simulink model "Ten_phase_nine_leg_relocated_L3_L7"  (R2025b)
settings: Solver=VariableStepAuto  StartTime=0.0  StopTime=0.05  FixedStep=1e-6  MaxStep=1e-6  RelTol=1e-4
values from neighbouring files (symbols this model uses):
  bias_current = 5    [parameters_for_AMB_topology.m]
  half_SW_Ts = SW_Ts*0.5    (= 2.5e-05)    [parameters_for_AMB_topology.m]
  K_i = 2*pi*f_c*R_value/U_dc    (= 47.1238898038)    [parameters_for_AMB_topology.m]
  K_p = 2*pi*f_c*L_value/U_dc    (= 0.0235619449019)    [parameters_for_AMB_topology.m]
  R_value = 1    [parameters_for_AMB_topology.m]
  SW_Ts = 1/(SW_frequency)    (= 5e-05)    [parameters_for_AMB_topology.m]
libraries: fl_lib x61, simulink x39, nesl_utility x29, eeGeneralControl x28, ee_lib x19
(part 1 of 4)
settings Model: SimulationMode=accelerator  Creator=ubuntu  LastModifiedBy=ubuntu

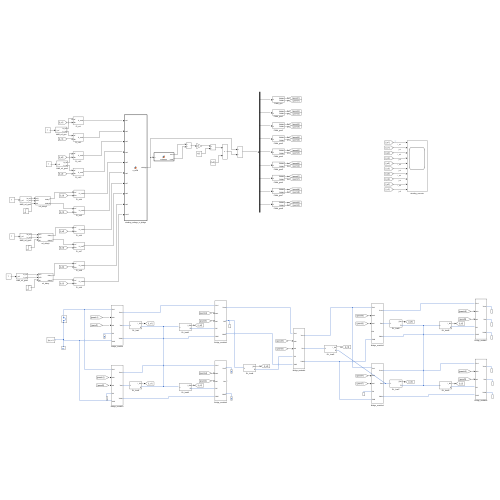
[thumbnail: Simulink's stored preview of the top-level diagram]
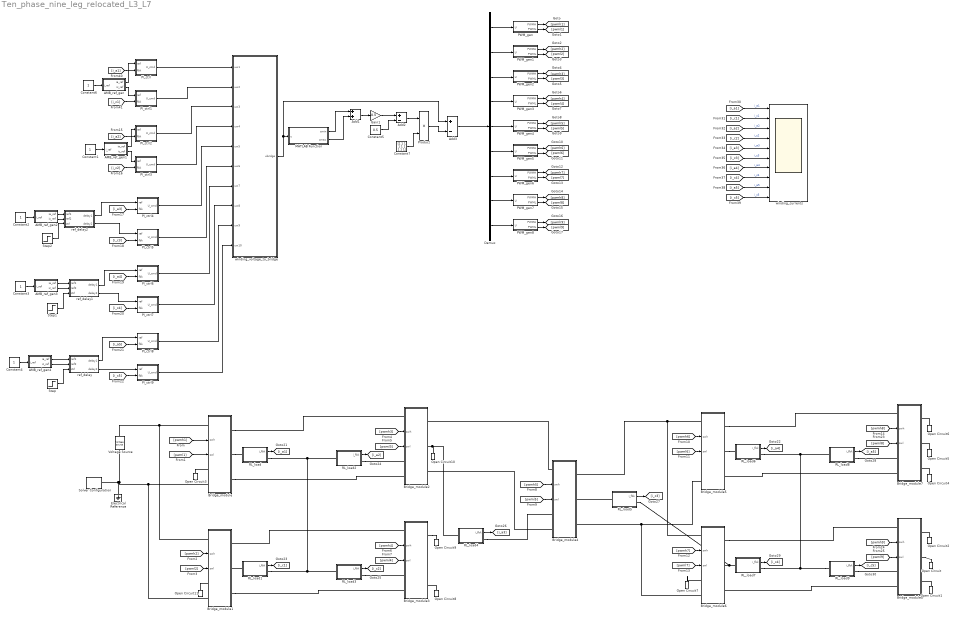
== system Ten_phase_nine_leg_relocated_L3_L7 ==
  AMB_ref_gen : Subsystem
  AMB_ref_gen1 : Subsystem
  AMB_ref_gen2 : Subsystem
  AMB_ref_gen3 : Subsystem
  AMB_ref_gen4 : Subsystem
  Add1 : Sum
  Add2 : Sum  Inputs=+-
  Add3 : Sum  Inputs=+-
  Bridge_module : Subsystem
      settings: PortSchema="{\"entries\":[{\"content\":{\"sides\":[{\"content\":{\"connectorIds\":[\"LConn1\",\"In1\",\"In2\",\"LConn2\",\"LConn3\"]},\"type\":\"ConnectorPlacement.EquallySpacedRectSide\",\"uuid\":\"d53b2940-a672-44eb-b8dc-5a9e6180756a\"},{\"content\":{\"connectorIds\":[\"RConn1\",\"RConn2\",\"RConn3\"],\"side\":\"RIGHT\"},\"type\":\"ConnectorPlacement.EquallySpacedRectSide\",\"uuid\":\"c4e7a2ca-919a-44db-8da7-3bac39d44d51\"},{\"content\":{\"side\":\"TOP\"},\"type\":\"ConnectorPlacement.EquallySpacedRectSide\",\"uuid\":\"b6113aa5-412c-49ab-b296-5158e67c3ca8\"}]},\"type\":\"ConnectorPlacement.EquallySpacedConnector\",\"uuid\":\"7447e388-299b-4a6a-b1b3-3d6a05a16289\"}],\"packageUris\":[\"http://schema.mathworks.com/mf0/Connector/R2020b\"],\"version\":\"1.0\"}"
  Bridge_module1 : Subsystem
      settings: PortSchema="{\"entries\":[{\"content\":{\"sides\":[{\"content\":{\"connectorIds\":[\"LConn1\",\"In1\",\"In2\",\"LConn2\",\"LConn3\"]},\"type\":\"ConnectorPlacement.EquallySpacedRectSide\",\"uuid\":\"d53b2940-a672-44eb-b8dc-5a9e6180756a\"},{\"content\":{\"connectorIds\":[\"RConn1\",\"RConn2\",\"RConn3\"],\"side\":\"RIGHT\"},\"type\":\"ConnectorPlacement.EquallySpacedRectSide\",\"uuid\":\"c4e7a2ca-919a-44db-8da7-3bac39d44d51\"},{\"content\":{\"side\":\"TOP\"},\"type\":\"ConnectorPlacement.EquallySpacedRectSide\",\"uuid\":\"b6113aa5-412c-49ab-b296-5158e67c3ca8\"}]},\"type\":\"ConnectorPlacement.EquallySpacedConnector\",\"uuid\":\"7447e388-299b-4a6a-b1b3-3d6a05a16289\"}],\"packageUris\":[\"http://schema.mathworks.com/mf0/Connector/R2020b\"],\"version\":\"1.0\"}"
  Bridge_module2 : Subsystem
      settings: PortSchema="{\"entries\":[{\"content\":{\"sides\":[{\"content\":{\"connectorIds\":[\"LConn1\",\"In1\",\"In2\",\"LConn2\",\"LConn3\"]},\"type\":\"ConnectorPlacement.EquallySpacedRectSide\",\"uuid\":\"d53b2940-a672-44eb-b8dc-5a9e6180756a\"},{\"content\":{\"connectorIds\":[\"RConn1\",\"RConn2\",\"RConn3\"],\"side\":\"RIGHT\"},\"type\":\"ConnectorPlacement.EquallySpacedRectSide\",\"uuid\":\"c4e7a2ca-919a-44db-8da7-3bac39d44d51\"},{\"content\":{\"side\":\"TOP\"},\"type\":\"ConnectorPlacement.EquallySpacedRectSide\",\"uuid\":\"b6113aa5-412c-49ab-b296-5158e67c3ca8\"}]},\"type\":\"ConnectorPlacement.EquallySpacedConnector\",\"uuid\":\"7447e388-299b-4a6a-b1b3-3d6a05a16289\"}],\"packageUris\":[\"http://schema.mathworks.com/mf0/Connector/R2020b\"],\"version\":\"1.0\"}"
  Bridge_module3 : Subsystem
      settings: PortSchema="{\"entries\":[{\"content\":{\"sides\":[{\"content\":{\"connectorIds\":[\"LConn1\",\"In1\",\"In2\",\"LConn2\",\"LConn3\"]},\"type\":\"ConnectorPlacement.EquallySpacedRectSide\",\"uuid\":\"d53b2940-a672-44eb-b8dc-5a9e6180756a\"},{\"content\":{\"connectorIds\":[\"RConn1\",\"RConn2\",\"RConn3\"],\"side\":\"RIGHT\"},\"type\":\"ConnectorPlacement.EquallySpacedRectSide\",\"uuid\":\"c4e7a2ca-919a-44db-8da7-3bac39d44d51\"},{\"content\":{\"side\":\"TOP\"},\"type\":\"ConnectorPlacement.EquallySpacedRectSide\",\"uuid\":\"b6113aa5-412c-49ab-b296-5158e67c3ca8\"}]},\"type\":\"ConnectorPlacement.EquallySpacedConnector\",\"uuid\":\"7447e388-299b-4a6a-b1b3-3d6a05a16289\"}],\"packageUris\":[\"http://schema.mathworks.com/mf0/Connector/R2020b\"],\"version\":\"1.0\"}"
  Bridge_module4 : Subsystem
      settings: PortSchema="{\"entries\":[{\"content\":{\"sides\":[{\"content\":{\"connectorIds\":[\"LConn1\",\"In1\",\"In2\",\"LConn2\",\"LConn3\"]},\"type\":\"ConnectorPlacement.EquallySpacedRectSide\",\"uuid\":\"d53b2940-a672-44eb-b8dc-5a9e6180756a\"},{\"content\":{\"connectorIds\":[\"RConn1\",\"RConn2\",\"RConn3\"],\"side\":\"RIGHT\"},\"type\":\"ConnectorPlacement.EquallySpacedRectSide\",\"uuid\":\"c4e7a2ca-919a-44db-8da7-3bac39d44d51\"},{\"content\":{\"side\":\"TOP\"},\"type\":\"ConnectorPlacement.EquallySpacedRectSide\",\"uuid\":\"b6113aa5-412c-49ab-b296-5158e67c3ca8\"}]},\"type\":\"ConnectorPlacement.EquallySpacedConnector\",\"uuid\":\"7447e388-299b-4a6a-b1b3-3d6a05a16289\"}],\"packageUris\":[\"http://schema.mathworks.com/mf0/Connector/R2020b\"],\"version\":\"1.0\"}"
  Bridge_module5 : Subsystem
      settings: PortSchema="{\"entries\":[{\"content\":{\"sides\":[{\"content\":{\"connectorIds\":[\"LConn1\",\"In1\",\"In2\",\"LConn2\",\"LConn3\"]},\"type\":\"ConnectorPlacement.EquallySpacedRectSide\",\"uuid\":\"d53b2940-a672-44eb-b8dc-5a9e6180756a\"},{\"content\":{\"connectorIds\":[\"RConn1\",\"RConn2\",\"RConn3\"],\"side\":\"RIGHT\"},\"type\":\"ConnectorPlacement.EquallySpacedRectSide\",\"uuid\":\"c4e7a2ca-919a-44db-8da7-3bac39d44d51\"},{\"content\":{\"side\":\"TOP\"},\"type\":\"ConnectorPlacement.EquallySpacedRectSide\",\"uuid\":\"b6113aa5-412c-49ab-b296-5158e67c3ca8\"}]},\"type\":\"ConnectorPlacement.EquallySpacedConnector\",\"uuid\":\"7447e388-299b-4a6a-b1b3-3d6a05a16289\"}],\"packageUris\":[\"http://schema.mathworks.com/mf0/Connector/R2020b\"],\"version\":\"1.0\"}"
  Bridge_module6 : Subsystem
      settings: PortSchema="{\"entries\":[{\"content\":{\"sides\":[{\"content\":{\"connectorIds\":[\"LConn1\",\"In1\",\"In2\",\"LConn2\",\"LConn3\"]},\"type\":\"ConnectorPlacement.EquallySpacedRectSide\",\"uuid\":\"d53b2940-a672-44eb-b8dc-5a9e6180756a\"},{\"content\":{\"connectorIds\":[\"RConn1\",\"RConn2\",\"RConn3\"],\"side\":\"RIGHT\"},\"type\":\"ConnectorPlacement.EquallySpacedRectSide\",\"uuid\":\"c4e7a2ca-919a-44db-8da7-3bac39d44d51\"},{\"content\":{\"side\":\"TOP\"},\"type\":\"ConnectorPlacement.EquallySpacedRectSide\",\"uuid\":\"b6113aa5-412c-49ab-b296-5158e67c3ca8\"}]},\"type\":\"ConnectorPlacement.EquallySpacedConnector\",\"uuid\":\"7447e388-299b-4a6a-b1b3-3d6a05a16289\"}],\"packageUris\":[\"http://schema.mathworks.com/mf0/Connector/R2020b\"],\"version\":\"1.0\"}"
  Bridge_module7 : Subsystem
      settings: PortSchema="{\"entries\":[{\"content\":{\"sides\":[{\"content\":{\"connectorIds\":[\"LConn1\",\"In1\",\"In2\",\"LConn2\",\"LConn3\"]},\"type\":\"ConnectorPlacement.EquallySpacedRectSide\",\"uuid\":\"d53b2940-a672-44eb-b8dc-5a9e6180756a\"},{\"content\":{\"connectorIds\":[\"RConn1\",\"RConn2\",\"RConn3\"],\"side\":\"RIGHT\"},\"type\":\"ConnectorPlacement.EquallySpacedRectSide\",\"uuid\":\"c4e7a2ca-919a-44db-8da7-3bac39d44d51\"},{\"content\":{\"side\":\"TOP\"},\"type\":\"ConnectorPlacement.EquallySpacedRectSide\",\"uuid\":\"b6113aa5-412c-49ab-b296-5158e67c3ca8\"}]},\"type\":\"ConnectorPlacement.EquallySpacedConnector\",\"uuid\":\"7447e388-299b-4a6a-b1b3-3d6a05a16289\"}],\"packageUris\":[\"http://schema.mathworks.com/mf0/Connector/R2020b\"],\"version\":\"1.0\"}"
  Bridge_module8 : Subsystem
      settings: PortSchema="{\"entries\":[{\"content\":{\"sides\":[{\"content\":{\"connectorIds\":[\"LConn1\",\"In1\",\"In2\",\"LConn2\",\"LConn3\"]},\"type\":\"ConnectorPlacement.EquallySpacedRectSide\",\"uuid\":\"d53b2940-a672-44eb-b8dc-5a9e6180756a\"},{\"content\":{\"connectorIds\":[\"RConn1\",\"RConn2\",\"RConn3\"],\"side\":\"RIGHT\"},\"type\":\"ConnectorPlacement.EquallySpacedRectSide\",\"uuid\":\"c4e7a2ca-919a-44db-8da7-3bac39d44d51\"},{\"content\":{\"side\":\"TOP\"},\"type\":\"ConnectorPlacement.EquallySpacedRectSide\",\"uuid\":\"b6113aa5-412c-49ab-b296-5158e67c3ca8\"}]},\"type\":\"ConnectorPlacement.EquallySpacedConnector\",\"uuid\":\"7447e388-299b-4a6a-b1b3-3d6a05a16289\"}],\"packageUris\":[\"http://schema.mathworks.com/mf0/Connector/R2020b\"],\"version\":\"1.0\"}"
  Constant{1..4,6} (5 alike) : Constant
  Constant5 : Constant  Value=0.5
  Constant7 : Constant  Value=[1 1 1 1 1 1 1 1 1]
  Demux : Demux  Outputs=9
  Electrical Reference : fl_lib/Electrical/Electrical Elements/Electrical Reference
  Gain1 : Gain  Gain=0.5
  MATLAB Function : MATLAB Function  TreatAsAtomicUnit=on
  Open Circuit{,1..11} (12 alike) : fl_lib/Electrical/Electrical Elements/Open Circuit  v_specify=off  v_priority=None  v=0 V  v_nominal_specify=off  v_nominal_value=1  v_nominal_unit=V
  PI_ctrl : Subsystem
  PI_ctrl1 : Subsystem
  PI_ctrl2 : Subsystem
  PI_ctrl3 : Subsystem
  PI_ctrl4 : Subsystem
  PI_ctrl5 : Subsystem
  PI_ctrl6 : Subsystem
  PI_ctrl7 : Subsystem
  PI_ctrl8 : Subsystem
  PI_ctrl9 : Subsystem
  PWM_gen : Subsystem
  PWM_gen1 : Subsystem
  PWM_gen2 : Subsystem
  PWM_gen3 : Subsystem
  PWM_gen4 : Subsystem
  PWM_gen5 : Subsystem
  PWM_gen6 : Subsystem
  PWM_gen7 : Subsystem
  PWM_gen8 : Subsystem
  Product : Product
  RL_load : Subsystem
  RL_load1 : Subsystem
  RL_load2 : Subsystem
  RL_load3 : Subsystem
  RL_load4 : Subsystem
  RL_load5 : Subsystem
  RL_load6 : Subsystem
  RL_load7 : Subsystem
  RL_load8 : Subsystem
  RL_load9 : Subsystem
  Solver Configuration : nesl_utility/Solver Configuration  PhysicalDomain=network_engine_domain  SubClassName=solver  LeftPortType=input  RightPortType=generic  Tones=[]  Harmonics=[]  SimulateNoise=off  Profile=off  UseLocalSampling=off  EnableSwitchedLinearOptims=on  FrequencyDomain=off  UseCCode=off  RelTol=0.001  AbsTol=0.001  MinStep=1e-09  ToWorkspace=off  RevertToSquareIcSolve=off  NumHomotopyIterations=100  PhasorMode=off  PhasorModeNumHarmonics=1  ConsistencySolver=NEWTON_XTOL_AFTER_FTOL  IndexReductionMethod=DerivativeReplacement  DoDC=off  ResidualTolerance=1e-09  ConsistencyTolSource=GLOBAL  ConsistencyAbsTol=0.001  ConsistencyRelTol=0.001  ConsistencyTolFactor=0.001  UseLocalSolver=off  LocalSolverChoice=NE_TRAPEZOIDAL_ADVANCER  ResolveIndetEquations=on  FunctionEvalNumThread=1  LocalSolverSampleTime=1e-8  DoFixedCost=off  MaxNonlinIter=3  MaxModeIter=2  ComputeImpulses=off  ImpulseIterations=2  LinearAlgebra=auto  LinearAlgebraNumThread=0  EquationFormulation=NE_TIME_EF  DelaysMemoryBudget=1024  AutomaticFiltering=on  FilteringTimeConstant=0.001  PartitionStorageMethod=AS_NEEDED  PartitionMemoryBudget=1024  PartitionMethod=ROBUST  MultibodyUseLocalSolver=off  MultibodyLocalSolverChoice=ODE1  MultibodyLocalSolverSampleTime=0.001
  Step : Step  Time=0.001*2  SampleTime=0
  Step1 : Step  Time=0.001*2  SampleTime=0
  Step2 : Step  Time=0.001*4  SampleTime=0
  Voltage Source : ee_lib/Sources/Voltage Source  dc_voltage=U_dc V  ac_voltage=0 V  ac_shift=0 rad  ac_frequency=60 Hz  noise_mode=ee.enum.sources.noise.Disabled  PSD=0 V^2/Hz  sample_time=1e-3 s  repeatability=ee.enum.sources.repeatability.NotRepeatable  user_seed=0  auto_seed=3499211588  i_specify=off  i_priority=None  i=0 A  i_nominal_specify=off  i_nominal_value=1  i_nominal_unit=A  v_specify=off  v_priority=None  v=0 V  v_nominal_specify=off  v_nominal_value=1  v_nominal_unit=V
  ref_delay : Subsystem
  ref_delay1 : Subsystem
  ref_delay2 : Subsystem
  winding_currents : Scope  NumInputPorts=10
      settings: ActiveDisplayYMinimum=-0.75203082398024912  ActiveDisplayYMaximum=6.6524809321526215
  winding_voltage_to_bridge : MATLAB Function  TreatAsAtomicUnit=on
  wires:
  [i_a1] -> winding_currents/1  "i_a1"
  [i_c1] -> winding_currents/2  "i_c1"
  [i_a2] -> winding_currents/3  "i_a2"
  [i_c2] -> winding_currents/4  "i_c2"
  [i_a3] -> winding_currents/5  "i_a3"
  [i_c3] -> winding_currents/6  "i_c3"
  [i_a4] -> winding_currents/7  "i_a4"
  [i_c4] -> winding_currents/8  "i_c4"
  [i_a5] -> winding_currents/9  "i_a5"
  [i_c5] -> winding_currents/10  "i_c5"
  AMB_ref_gen/1(ia_ref) -> PI_ctrl/1(ref)
  AMB_ref_gen/2(ic_ref) -> PI_ctrl1/1(ref)
  Constant6/1 -> AMB_ref_gen/1(i_ref)
  [i_a1] -> PI_ctrl/2(fbk)
  [i_c1] -> PI_ctrl1/2(fbk)
  [i_c2] -> PI_ctrl3/2(fbk)
  [i_a2] -> PI_ctrl2/2(fbk)
  Constant1/1 -> AMB_ref_gen1/1(i_ref)
  [i_c3] -> PI_ctrl5/2(fbk)
  [i_a3] -> PI_ctrl4/2(fbk)
  Constant2/1 -> AMB_ref_gen2/1(i_ref)
  [i_c4] -> PI_ctrl7/2(fbk)
  [i_a4] -> PI_ctrl6/2(fbk)
  Constant3/1 -> AMB_ref_gen3/1(i_ref)
  [i_c5] -> PI_ctrl9/2(fbk)
  Constant4/1 -> AMB_ref_gen4/1(i_ref)
  [i_a5] -> PI_ctrl8/2(fbk)
  MATLAB Function/1(cmin) -> Add1/1
  MATLAB Function/2(cmax) -> Add1/2
  Add1/1 -> Gain1/1
  Gain1/1 -> Add2/1
  Constant5/1 -> Add2/2
  Add2/1 -> Product/1
  Constant7/1 -> Product/2
  Product/1 -> Add3/2
  Add3/1 -> Demux/1
  Demux/7 -> PWM_gen6/1(U)
  Demux/8 -> PWM_gen7/1(U)
  Demux/9 -> PWM_gen8/1(U)
  Demux/6 -> PWM_gen5/1(U)
  Demux/1 -> PWM_gen/1(U)
  Demux/2 -> PWM_gen1/1(U)
  Demux/3 -> PWM_gen2/1(U)
  Demux/4 -> PWM_gen3/1(U)
  Demux/5 -> PWM_gen4/1(U)
  RL_load/1(i_fbk) -> [i_a1]
  winding_voltage_to_bridge/1(ubridge) -> Add3/1, MATLAB Function/1(u)
  PWM_gen/1(PWMH) -> [pwmh1]
  PWM_gen/2(PWML) -> [pwml1]
  PWM_gen1/1(PWMH) -> [pwmh2]
  PWM_gen1/2(PWML) -> [pwml2]
  PWM_gen2/1(PWMH) -> [pwmh3]
  PWM_gen2/2(PWML) -> [pwml3]
  PWM_gen3/1(PWMH) -> [pwmh4]
  PWM_gen3/2(PWML) -> [pwml4]
  PWM_gen4/1(PWMH) -> [pwmh5]
  PWM_gen4/2(PWML) -> [pwml5]
  PWM_gen5/1(PWMH) -> [pwmh6]
  PWM_gen5/2(PWML) -> [pwml6]
  PWM_gen6/1(PWMH) -> [pwmh7]
  PWM_gen6/2(PWML) -> [pwml7]
  PWM_gen7/1(PWMH) -> [pwmh8]
  PWM_gen7/2(PWML) -> [pwml8]
  PWM_gen8/1(PWMH) -> [pwmh9]
  PWM_gen8/2(PWML) -> [pwml9]
  [pwml1] -> Bridge_module/2(swl)
  [pwmh1] -> Bridge_module/1(swh)
  AMB_ref_gen4/2(ic_ref) -> ref_delay/2(ref2)
  AMB_ref_gen4/1(ia_ref) -> ref_delay/1(ref1)
  ref_delay/1(delay1) -> PI_ctrl8/1(ref)
  ref_delay/2(delay2) -> PI_ctrl9/1(ref)
  Step/1 -> ref_delay/3(ctrl)
  Step1/1 -> ref_delay1/3(ctrl)
  Step2/1 -> ref_delay2/3(ctrl)
  AMB_ref_gen3/1(ia_ref) -> ref_delay1/1(ref1)
  AMB_ref_gen3/2(ic_ref) -> ref_delay1/2(ref2)
  ref_delay1/1(delay1) -> PI_ctrl6/1(ref)
  ref_delay1/2(delay2) -> PI_ctrl7/1(ref)
  ref_delay2/2(delay2) -> PI_ctrl5/1(ref)
  ref_delay2/1(delay1) -> PI_ctrl4/1(ref)
  AMB_ref_gen2/1(ia_ref) -> ref_delay2/1(ref1)
  AMB_ref_gen2/2(ic_ref) -> ref_delay2/2(ref2)
  AMB_ref_gen1/2(ic_ref) -> PI_ctrl3/1(ref)
  AMB_ref_gen1/1(ia_ref) -> PI_ctrl2/1(ref)
  RL_load6/1(i_fbk) -> [i_a4]
  RL_load1/1(i_fbk) -> [i_c1]
  RL_load2/1(i_fbk) -> [i_a2]
  RL_load3/1(i_fbk) -> [i_c2]
  RL_load4/1(i_fbk) -> [i_a3]
  RL_load5/1(i_fbk) -> [i_c3]
  RL_load7/1(i_fbk) -> [i_c4]
  RL_load8/1(i_fbk) -> [i_a5]
  RL_load9/1(i_fbk) -> [i_c5]
  PI_ctrl/1(U_cmd) -> winding_voltage_to_bridge/1(uw1)
  PI_ctrl1/1(U_cmd) -> winding_voltage_to_bridge/2(uw2)
  PI_ctrl2/1(U_cmd) -> winding_voltage_to_bridge/3(uw3)
  PI_ctrl3/1(U_cmd) -> winding_voltage_to_bridge/4(uw4)
  PI_ctrl4/1(U_cmd) -> winding_voltage_to_bridge/5(uw5)
  PI_ctrl5/1(U_cmd) -> winding_voltage_to_bridge/6(uw6)
  PI_ctrl6/1(U_cmd) -> winding_voltage_to_bridge/7(uw7)
  PI_ctrl7/1(U_cmd) -> winding_voltage_to_bridge/8(uw8)
  PI_ctrl8/1(U_cmd) -> winding_voltage_to_bridge/9(uw9)
  PI_ctrl9/1(U_cmd) -> winding_voltage_to_bridge/10(uw10)
  [pwmh5] -> Bridge_module4/1(swh)
  [pwml5] -> Bridge_module4/2(swl)
  [pwml2] -> Bridge_module1/2(swl)
  [pwmh2] -> Bridge_module1/1(swh)
  [pwml3] -> Bridge_module2/2(swl)
  [pwmh3] -> Bridge_module2/1(swh)
  [pwml4] -> Bridge_module3/2(swl)
  [pwmh4] -> Bridge_module3/1(swh)
  [pwml6] -> Bridge_module5/2(swl)
  [pwmh6] -> Bridge_module5/1(swh)
  [pwml7] -> Bridge_module6/2(swl)
  [pwmh7] -> Bridge_module6/1(swh)
  [pwml8] -> Bridge_module7/2(swl)
  [pwmh8] -> Bridge_module7/1(swh)
  [pwml9] -> Bridge_module8/2(swl)
  [pwmh9] -> Bridge_module8/1(swh)
  connections:
  Electrical Reference/LConn1 -- Bridge_module1/LConn3 -- Bridge_module/LConn3 -- Voltage Source/RConn1 -- Solver Configuration/RConn1
  Bridge_module/RConn2 -- RL_load/LConn1
  Bridge_module/LConn1 -- Bridge_module1/LConn1 -- Voltage Source/LConn1
  Bridge_module/LConn2 -- Open Circuit3/LConn1
  RL_load1/LConn1 -- Bridge_module1/RConn2
  RL_load1/RConn1 -- RL_load2/LConn1 -- RL_load/RConn1 -- RL_load3/LConn1
  RL_load2/RConn1 -- Bridge_module2/LConn2
  RL_load3/RConn1 -- Bridge_module3/LConn2
  RL_load9/LConn1 -- RL_load7/RConn1 -- RL_load8/LConn1 -- RL_load6/RConn1
  Bridge_module6/RConn2 -- RL_load7/LConn1 -- RL_load5/RConn1
  RL_load8/RConn1 -- Bridge_module7/LConn2
  Bridge_module5/RConn2 -- RL_load6/LConn1
  RL_load9/RConn1 -- Bridge_module8/LConn2
  RL_load5/LConn1 -- Bridge_module4/RConn2
  RL_load4/RConn1 -- Bridge_module4/LConn2
  Bridge_module/RConn1 -- Bridge_module2/LConn1
  Bridge_module/RConn3 -- Bridge_module2/LConn3
  Bridge_module3/LConn1 -- Bridge_module1/RConn1
  Bridge_module1/RConn3 -- Bridge_module3/LConn3
  Bridge_module4/LConn1 -- Bridge_module2/RConn1
  Bridge_module4/LConn3 -- Bridge_module2/RConn3
  Bridge_module5/LConn1 -- Bridge_module4/RConn1 -- Bridge_module6/LConn1
  Bridge_module5/LConn3 -- Bridge_module6/LConn3 -- Bridge_module4/RConn3
  Bridge_module5/RConn1 -- Bridge_module7/LConn1
  Bridge_module7/LConn3 -- Bridge_module5/RConn3
  Bridge_module6/RConn1 -- Bridge_module8/LConn1
  Bridge_module8/LConn3 -- Bridge_module6/RConn3
  Open Circuit1/LConn1 -- Bridge_module8/RConn3
  Bridge_module8/RConn2 -- Open Circuit/LConn1
  Open Circuit2/LConn1 -- Bridge_module8/RConn1
  Open Circuit5/LConn1 -- Bridge_module7/RConn2
  Open Circuit6/LConn1 -- Bridge_module7/RConn1
  Open Circuit4/LConn1 -- Bridge_module7/RConn3
  Open Circuit7/LConn1 -- Bridge_module6/LConn2
  Bridge_module3/RConn1 -- Open Circuit9/LConn1
  Open Circuit8/LConn1 -- Bridge_module3/RConn3
  Bridge_module2/RConn2 -- Open Circuit10/LConn1 -- RL_load4/LConn1
  Open Circuit11/LConn1 -- Bridge_module1/LConn2

== system Ten_phase_nine_leg_relocated_L3_L7/AMB_ref_gen ==
  i_ref : Inport
  Add : Sum
  Add1 : Sum  Inputs=-+
  Constant : Constant  Value=bias_current
  Gain : Gain  Gain=0.5
  ia_ref : Outport
  ic_ref : Outport  Port=2
  wires:
  i_ref/1 -> Gain/1
  Gain/1 -> Add1/1, Add/2
  Add/1 -> ia_ref/1
  Constant/1 -> Add1/2, Add/1
  Add1/1 -> ic_ref/1

== system Ten_phase_nine_leg_relocated_L3_L7/AMB_ref_gen1 ==
  i_ref : Inport
  Add : Sum
  Add1 : Sum  Inputs=-+
  Constant : Constant  Value=bias_current
  Gain : Gain  Gain=0.5
  ia_ref : Outport
  ic_ref : Outport  Port=2
  wires:
  i_ref/1 -> Gain/1
  Gain/1 -> Add1/1, Add/2
  Add/1 -> ia_ref/1
  Constant/1 -> Add1/2, Add/1
  Add1/1 -> ic_ref/1

== system Ten_phase_nine_leg_relocated_L3_L7/AMB_ref_gen2 ==
  i_ref : Inport
  Add : Sum
  Add1 : Sum  Inputs=-+
  Constant : Constant  Value=bias_current
  Gain : Gain  Gain=0.5
  ia_ref : Outport
  ic_ref : Outport  Port=2
  wires:
  i_ref/1 -> Gain/1
  Gain/1 -> Add1/1, Add/2
  Add/1 -> ia_ref/1
  Constant/1 -> Add1/2, Add/1
  Add1/1 -> ic_ref/1

== system Ten_phase_nine_leg_relocated_L3_L7/AMB_ref_gen3 ==
  i_ref : Inport
  Add : Sum
  Add1 : Sum  Inputs=-+
  Constant : Constant  Value=bias_current
  Gain : Gain  Gain=0.5
  ia_ref : Outport
  ic_ref : Outport  Port=2
  wires:
  i_ref/1 -> Gain/1
  Gain/1 -> Add1/1, Add/2
  Add/1 -> ia_ref/1
  Constant/1 -> Add1/2, Add/1
  Add1/1 -> ic_ref/1

== system Ten_phase_nine_leg_relocated_L3_L7/AMB_ref_gen4 ==
  i_ref : Inport
  Add : Sum
  Add1 : Sum  Inputs=-+
  Constant : Constant  Value=bias_current
  Gain : Gain  Gain=0.5
  ia_ref : Outport
  ic_ref : Outport  Port=2
  wires:
  i_ref/1 -> Gain/1
  Gain/1 -> Add1/1, Add/2
  Add/1 -> ia_ref/1
  Constant/1 -> Add1/2, Add/1
  Add1/1 -> ic_ref/1

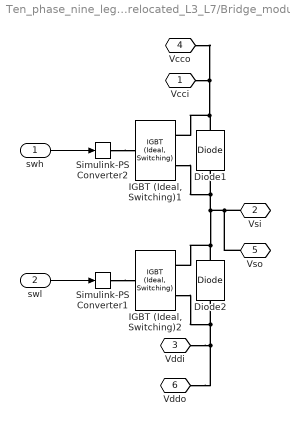
== system Ten_phase_nine_leg_relocated_L3_L7/Bridge_module ==
  swh : Inport
  swl : Inport  Port=2
  Diode1 : fl_lib/Electrical/Electrical Elements/Diode  Vf=0.6 V  Ron=0.3 Ohm  Goff=1e-8 1/Ohm  i_specify=off  i_priority=None  i=0 A  i_nominal_specify=off  i_nominal_value=1  i_nominal_unit=A  v_specify=off  v_priority=None  v=0 V  v_nominal_specify=off  v_nominal_value=1  v_nominal_unit=V
  Diode2 : fl_lib/Electrical/Electrical Elements/Diode  Vf=0.6 V  Ron=0.3 Ohm  Goff=1e-8 1/Ohm  i_specify=off  i_priority=None  i=0 A  i_nominal_specify=off  i_nominal_value=1  i_nominal_unit=A  v_specify=off  v_priority=None  v=0 V  v_nominal_specify=off  v_nominal_value=1  v_nominal_unit=V
  "IGBT (Ideal, Switching)1" : ee_lib/Semiconductors & Converters/IGBT (Ideal, Switching)  port_option=ee.enum.controlport.ps  Vf=0.8 V  Ron=0.001 Ohm  Goff=1e-5 1/Ohm  Vth=6 V  diode_param=ee.enum.semiconductors.protectionDiode.external  diode_Vf=0.8 V  diode_Ron=0.001 Ohm  diode_Goff=1e-5 1/Ohm  diode_C=50e-9 F  diode_iRM=-235 A  diode_iF=300 A  diode_idot=-50 A/us  diode_trr_param=ee.enum.converters.diodeReverseParam.trr_factor  diode_trr_factor=3  diode_trr=15 us  diode_Qrr=1500 s*uA  ice_specify=off  ice_priority=None  ice=0 A  ice_nominal_specify=off  ice_nominal_value=1  ice_nominal_unit=A  vce_specify=off  vce_priority=None  vce=0 V  vce_nominal_specify=off  vce_nominal_value=1  vce_nominal_unit=V  vge_specify=off  vge_priority=None  vge=0 V  vge_nominal_specify=off  vge_nominal_value=1  vge_nominal_unit=V  thermal_loss_option=ee.enum.converters.thermalLossOption.constantvalues  Von_data=[0, .1, .6, .8, 1, 1.3, 1.6, 2, 2.4; 0, .1, .7, 1, 1.2, 1.5, 1.9, 2.4, 2.8] V  Tj=[298.15, 398.15] K  Iout_data=[0, .1, 1, 5, 10, 20, 40, 70, 100] A  Eon_data=[0, .0024, .024, .12, .2, .48, 1.04, 2.16, 3.24; 0, .003, .03, .15, .25, .6, 1.3, 2.7, 4.05] * 1e-3 J  Eoff_data=[0, .0007, .0066, .033, .066, .17, .33, .83, 1.5; 0, .001, .01, .05, .1, .25, .5, 1.2, 2.2] * 1e-3 J  Eon_data_3D=[zeros(2, 9, 3)] J  Eoff_data_3D=[zeros(2, 9, 3)] J  Tj_loss=[298.15, 398.15] K  Iout_data_loss=[0, .1, 1, 5, 10, 20, 40, 70, 100] A  tabulateWithVce=false  Vce_loss=[0, 150, 300] V  Eon_scalar=22.86e-3 J  Eoff_scalar=17.14e-3 J  Voff=300 V  Iout_scalar=600 A  useCurrentFromPreviousCycle=false  useVoltageFromPreviousCycle=false  diodeModelType=ee.enum.converters.diodeModelType.pwl  diodeTableType=ee.enum.diode.tableType.IfMat  diode_ReverseIVType=ee.enum.diode.diodeReverseIV.constant  diode_IfMat=[.07, .12, .19, 1.75, 4.24, 7.32, 11.2; .16, .3, .72, 2.14, 4.02, 6.35, 9.12] A  diode_VfMat=[.9, 1.15, 1.25, 1.5, 1.75, 2.17, 2.6, 2.85; .58, .68, .75, 1.1, 1.38, 1.77, 2.27, 2.7] V  diode_TjVec=[25, 125] degC  diode_VfVec=[.5, .7, .9, 1.3, 1.7, 2.1, 2.5] V  diode_IfVec=[.1, .2, .5, 1, 2, 4, 7, 10] A  diode_IrMat=[1e-06, 2e-06, 5e-06, 1e-05, 2.5e-05, 5e-05, .0001; 2e-06, 5e-06, 1e-05, 4e-05, 8e-05, .0002, .0005] A  diode_VrMat=[10, 100, 200, 250, 300, 325, 350; 10, 70, 160, 220, 270, 300, 320] V  diode_VrVec=[10, 20, 40, 50, 70, 80, 100] V  diode_IrVec=[1e-06, 2e-06, 5e-06, 1e-05, 2e-05, 5e-05, .0001] A  diode_Vr=-600 V  diode_Ls=150 nH  diode_Erec=0.03 J  diode_rec_loss_model=ee.enum.diode.reverseRecoveryModel.fixed  diode_ErecVal=0 J  diode_scaleWithIandV=true  diode_ErecMat=zeros(2, 3) J  diode_TjrecVec=[298.15, 398.15] K  diode_IfrecVec=[.1, 1, 10] A  diode_IrecVal=10 A  diode_VrecVal=10 V  diode_tFilter=1 / 1000 / 100 s  separateThermalPortForDiode=false  thermal_network_parameterization=ee.enum.thermalNetworkTopology.external  Rth=[.08, .5] K/W  Rth_Cauer=[.08, .1, .5] K/W  Rth_Foster=[.08, .14, .22, .16] K/W  thermal_mass_parameterization=ee.enum.thermalNetwork.timeconstant  thermal_mass=[.01, .5] J/K  thermal_mass_Cauer=[.01, .1, .5] J/K  thermal_mass_Foster=[.001, .005, .05, .5] J/K  thermal_time_constant=[.001, .2] s  thermal_time_constant_Cauer=[.001, .1, .2] s  thermal_time_constant_Foster=[7e-05, .0007, .01, .08] s  thermal_mass_initial_temperatures=[25, 25] degC  thermal_mass_initial_temperatures_Cauer=[25, 25, 25] degC  junction_thermal_mass=0.01 J/K  Tvec_initial_Foster=[25, 25, 25, 25] degC  RthDiode=[.03, .2] K/W  RthCauerDiode=[.03, .1, .2] K/W  RthFosterDiode=[.03, .2] K/W  thermalMassDiode=[3, 25] J/K  thermalMassCauerDiode=[3, 10, 25] J/K  thermalMassFosterDiode=[33, 50] J/K  thermalTauDiode=[.1, 5] s  thermalTauCauerDiode=[.1, 1, 5] s  thermalTauFosterDiode=[1, 10] s  thermalMassInitTempDiode=[25, 25] degC  thermalMassInitTempCauerDiode=[25, 25, 25] degC  junctionthermalMassDiode=0.1 J/K  TVecInitialFosterDiode=[25, 25, 25, 25] degC  no_thermal_network=0  IGBT_junction_temperature_specify=off  IGBT_junction_temperature_priority=None  IGBT_junction_temperature=25 degC  IGBT_junction_temperature_nominal_specify=off  IGBT_junction_temperature_nominal_value=1  IGBT_junction_temperature_nominal_unit=degC  diode_junction_temperature_specify=off  diode_junction_temperature_priority=None  diode_junction_temperature=25 degC  diode_junction_temperature_nominal_specify=off  diode_junction_temperature_nominal_value=1  diode_junction_temperature_nominal_unit=degC  Qj_specify=off  Qj_priority=None  Qj=0 W  Qj_nominal_specify=off  Qj_nominal_value=1  Qj_nominal_unit=W  accumulatedSwitchingLosses_specify=off  accumulatedSwitchingLosses_priority=None  accumulatedSwitchingLosses=0 J
  "IGBT (Ideal, Switching)2" : ee_lib/Semiconductors & Converters/IGBT (Ideal, Switching)  port_option=ee.enum.controlport.ps  Vf=0.8 V  Ron=0.001 Ohm  Goff=1e-5 1/Ohm  Vth=6 V  diode_param=ee.enum.semiconductors.protectionDiode.external  diode_Vf=0.8 V  diode_Ron=0.001 Ohm  diode_Goff=1e-5 1/Ohm  diode_C=50e-9 F  diode_iRM=-235 A  diode_iF=300 A  diode_idot=-50 A/us  diode_trr_param=ee.enum.converters.diodeReverseParam.trr_factor  diode_trr_factor=3  diode_trr=15 us  diode_Qrr=1500 s*uA  ice_specify=off  ice_priority=None  ice=0 A  ice_nominal_specify=off  ice_nominal_value=1  ice_nominal_unit=A  vce_specify=off  vce_priority=None  vce=0 V  vce_nominal_specify=off  vce_nominal_value=1  vce_nominal_unit=V  vge_specify=off  vge_priority=None  vge=0 V  vge_nominal_specify=off  vge_nominal_value=1  vge_nominal_unit=V  thermal_loss_option=ee.enum.converters.thermalLossOption.constantvalues  Von_data=[0, .1, .6, .8, 1, 1.3, 1.6, 2, 2.4; 0, .1, .7, 1, 1.2, 1.5, 1.9, 2.4, 2.8] V  Tj=[298.15, 398.15] K  Iout_data=[0, .1, 1, 5, 10, 20, 40, 70, 100] A  Eon_data=[0, .0024, .024, .12, .2, .48, 1.04, 2.16, 3.24; 0, .003, .03, .15, .25, .6, 1.3, 2.7, 4.05] * 1e-3 J  Eoff_data=[0, .0007, .0066, .033, .066, .17, .33, .83, 1.5; 0, .001, .01, .05, .1, .25, .5, 1.2, 2.2] * 1e-3 J  Eon_data_3D=[zeros(2, 9, 3)] J  Eoff_data_3D=[zeros(2, 9, 3)] J  Tj_loss=[298.15, 398.15] K  Iout_data_loss=[0, .1, 1, 5, 10, 20, 40, 70, 100] A  tabulateWithVce=false  Vce_loss=[0, 150, 300] V  Eon_scalar=22.86e-3 J  Eoff_scalar=17.14e-3 J  Voff=300 V  Iout_scalar=600 A  useCurrentFromPreviousCycle=false  useVoltageFromPreviousCycle=false  diodeModelType=ee.enum.converters.diodeModelType.pwl  diodeTableType=ee.enum.diode.tableType.IfMat  diode_ReverseIVType=ee.enum.diode.diodeReverseIV.constant  diode_IfMat=[.07, .12, .19, 1.75, 4.24, 7.32, 11.2; .16, .3, .72, 2.14, 4.02, 6.35, 9.12] A  diode_VfMat=[.9, 1.15, 1.25, 1.5, 1.75, 2.17, 2.6, 2.85; .58, .68, .75, 1.1, 1.38, 1.77, 2.27, 2.7] V  diode_TjVec=[25, 125] degC  diode_VfVec=[.5, .7, .9, 1.3, 1.7, 2.1, 2.5] V  diode_IfVec=[.1, .2, .5, 1, 2, 4, 7, 10] A  diode_IrMat=[1e-06, 2e-06, 5e-06, 1e-05, 2.5e-05, 5e-05, .0001; 2e-06, 5e-06, 1e-05, 4e-05, 8e-05, .0002, .0005] A  diode_VrMat=[10, 100, 200, 250, 300, 325, 350; 10, 70, 160, 220, 270, 300, 320] V  diode_VrVec=[10, 20, 40, 50, 70, 80, 100] V  diode_IrVec=[1e-06, 2e-06, 5e-06, 1e-05, 2e-05, 5e-05, .0001] A  diode_Vr=-600 V  diode_Ls=150 nH  diode_Erec=0.03 J  diode_rec_loss_model=ee.enum.diode.reverseRecoveryModel.fixed  diode_ErecVal=0 J  diode_scaleWithIandV=true  diode_ErecMat=zeros(2, 3) J  diode_TjrecVec=[298.15, 398.15] K  diode_IfrecVec=[.1, 1, 10] A  diode_IrecVal=10 A  diode_VrecVal=10 V  diode_tFilter=1 / 1000 / 100 s  separateThermalPortForDiode=false  thermal_network_parameterization=ee.enum.thermalNetworkTopology.external  Rth=[.08, .5] K/W  Rth_Cauer=[.08, .1, .5] K/W  Rth_Foster=[.08, .14, .22, .16] K/W  thermal_mass_parameterization=ee.enum.thermalNetwork.timeconstant  thermal_mass=[.01, .5] J/K  thermal_mass_Cauer=[.01, .1, .5] J/K  thermal_mass_Foster=[.001, .005, .05, .5] J/K  thermal_time_constant=[.001, .2] s  thermal_time_constant_Cauer=[.001, .1, .2] s  thermal_time_constant_Foster=[7e-05, .0007, .01, .08] s  thermal_mass_initial_temperatures=[25, 25] degC  thermal_mass_initial_temperatures_Cauer=[25, 25, 25] degC  junction_thermal_mass=0.01 J/K  Tvec_initial_Foster=[25, 25, 25, 25] degC  RthDiode=[.03, .2] K/W  RthCauerDiode=[.03, .1, .2] K/W  RthFosterDiode=[.03, .2] K/W  thermalMassDiode=[3, 25] J/K  thermalMassCauerDiode=[3, 10, 25] J/K  thermalMassFosterDiode=[33, 50] J/K  thermalTauDiode=[.1, 5] s  thermalTauCauerDiode=[.1, 1, 5] s  thermalTauFosterDiode=[1, 10] s  thermalMassInitTempDiode=[25, 25] degC  thermalMassInitTempCauerDiode=[25, 25, 25] degC  junctionthermalMassDiode=0.1 J/K  TVecInitialFosterDiode=[25, 25, 25, 25] degC  no_thermal_network=0  IGBT_junction_temperature_specify=off  IGBT_junction_temperature_priority=None  IGBT_junction_temperature=25 degC  IGBT_junction_temperature_nominal_specify=off  IGBT_junction_temperature_nominal_value=1  IGBT_junction_temperature_nominal_unit=degC  diode_junction_temperature_specify=off  diode_junction_temperature_priority=None  diode_junction_temperature=25 degC  diode_junction_temperature_nominal_specify=off  diode_junction_temperature_nominal_value=1  diode_junction_temperature_nominal_unit=degC  Qj_specify=off  Qj_priority=None  Qj=0 W  Qj_nominal_specify=off  Qj_nominal_value=1  Qj_nominal_unit=W  accumulatedSwitchingLosses_specify=off  accumulatedSwitchingLosses_priority=None  accumulatedSwitchingLosses=0 J
  Simulink-PS Converter1 : nesl_utility/Simulink-PS Converter  PhysicalDomain=network_engine_domain  SubClassName=ps_input  LeftPortType=input  RightPortType=output  PseudoPeriodic=off  Frequencies=[]  NoiseDistribution=none  NoiseParameters=[]  Unit=1  AffineConversion=off  FilteringAndDerivatives=provide  SimscapeFilterOrder=1  InputFilterTimeConstant=0.001  UdotUserProvided=0
  Simulink-PS Converter2 : nesl_utility/Simulink-PS Converter  PhysicalDomain=network_engine_domain  SubClassName=ps_input  LeftPortType=input  RightPortType=output  PseudoPeriodic=off  Frequencies=[]  NoiseDistribution=none  NoiseParameters=[]  Unit=1  AffineConversion=off  FilteringAndDerivatives=provide  SimscapeFilterOrder=1  InputFilterTimeConstant=0.001  UdotUserProvided=0
  Vcci : PMIOPort  Side=Left
  Vsi : PMIOPort  Port=2  Side=Left
  Vddi : PMIOPort  Port=3  Side=Left
  Vcco : PMIOPort  Port=4  Side=Right
  Vso : PMIOPort  Port=5  Side=Right
  Vddo : PMIOPort  Port=6  Side=Right
  wires:
  swh/1 -> Simulink-PS Converter2/1
  swl/1 -> Simulink-PS Converter1/1
  connections:
  Diode1/RConn1 -- Vcco/RConn1 -- Vcci/RConn1 -- "IGBT (Ideal, Switching)1"/RConn1
  Simulink-PS Converter2/RConn1 -- "IGBT (Ideal, Switching)1"/LConn1
  "IGBT (Ideal, Switching)1"/RConn2 -- Vso/RConn1 -- Vsi/RConn1 -- "IGBT (Ideal, Switching)2"/RConn1 -- Diode2/RConn1 -- Diode1/LConn1
  "IGBT (Ideal, Switching)2"/RConn2 -- Vddo/RConn1 -- Vddi/RConn1 -- Diode2/LConn1
  Simulink-PS Converter1/RConn1 -- "IGBT (Ideal, Switching)2"/LConn1

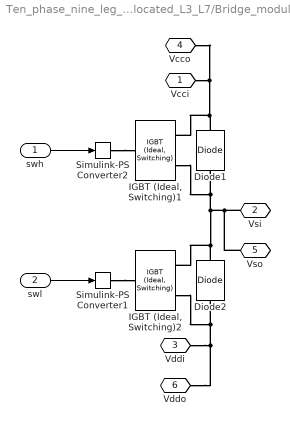
== system Ten_phase_nine_leg_relocated_L3_L7/Bridge_module1 ==
  swh : Inport
  swl : Inport  Port=2
  Diode1 : fl_lib/Electrical/Electrical Elements/Diode  Vf=0.6 V  Ron=0.3 Ohm  Goff=1e-8 1/Ohm  i_specify=off  i_priority=None  i=0 A  i_nominal_specify=off  i_nominal_value=1  i_nominal_unit=A  v_specify=off  v_priority=None  v=0 V  v_nominal_specify=off  v_nominal_value=1  v_nominal_unit=V
  Diode2 : fl_lib/Electrical/Electrical Elements/Diode  Vf=0.6 V  Ron=0.3 Ohm  Goff=1e-8 1/Ohm  i_specify=off  i_priority=None  i=0 A  i_nominal_specify=off  i_nominal_value=1  i_nominal_unit=A  v_specify=off  v_priority=None  v=0 V  v_nominal_specify=off  v_nominal_value=1  v_nominal_unit=V
  "IGBT (Ideal, Switching)1" : ee_lib/Semiconductors & Converters/IGBT (Ideal, Switching)  port_option=ee.enum.controlport.ps  Vf=0.8 V  Ron=0.001 Ohm  Goff=1e-5 1/Ohm  Vth=6 V  diode_param=ee.enum.semiconductors.protectionDiode.external  diode_Vf=0.8 V  diode_Ron=0.001 Ohm  diode_Goff=1e-5 1/Ohm  diode_C=50e-9 F  diode_iRM=-235 A  diode_iF=300 A  diode_idot=-50 A/us  diode_trr_param=ee.enum.converters.diodeReverseParam.trr_factor  diode_trr_factor=3  diode_trr=15 us  diode_Qrr=1500 s*uA  ice_specify=off  ice_priority=None  ice=0 A  ice_nominal_specify=off  ice_nominal_value=1  ice_nominal_unit=A  vce_specify=off  vce_priority=None  vce=0 V  vce_nominal_specify=off  vce_nominal_value=1  vce_nominal_unit=V  vge_specify=off  vge_priority=None  vge=0 V  vge_nominal_specify=off  vge_nominal_value=1  vge_nominal_unit=V  thermal_loss_option=ee.enum.converters.thermalLossOption.constantvalues  Von_data=[0, .1, .6, .8, 1, 1.3, 1.6, 2, 2.4; 0, .1, .7, 1, 1.2, 1.5, 1.9, 2.4, 2.8] V  Tj=[298.15, 398.15] K  Iout_data=[0, .1, 1, 5, 10, 20, 40, 70, 100] A  Eon_data=[0, .0024, .024, .12, .2, .48, 1.04, 2.16, 3.24; 0, .003, .03, .15, .25, .6, 1.3, 2.7, 4.05] * 1e-3 J  Eoff_data=[0, .0007, .0066, .033, .066, .17, .33, .83, 1.5; 0, .001, .01, .05, .1, .25, .5, 1.2, 2.2] * 1e-3 J  Eon_data_3D=[zeros(2, 9, 3)] J  Eoff_data_3D=[zeros(2, 9, 3)] J  Tj_loss=[298.15, 398.15] K  Iout_data_loss=[0, .1, 1, 5, 10, 20, 40, 70, 100] A  tabulateWithVce=false  Vce_loss=[0, 150, 300] V  Eon_scalar=22.86e-3 J  Eoff_scalar=17.14e-3 J  Voff=300 V  Iout_scalar=600 A  useCurrentFromPreviousCycle=false  useVoltageFromPreviousCycle=false  diodeModelType=ee.enum.converters.diodeModelType.pwl  diodeTableType=ee.enum.diode.tableType.IfMat  diode_ReverseIVType=ee.enum.diode.diodeReverseIV.constant  diode_IfMat=[.07, .12, .19, 1.75, 4.24, 7.32, 11.2; .16, .3, .72, 2.14, 4.02, 6.35, 9.12] A  diode_VfMat=[.9, 1.15, 1.25, 1.5, 1.75, 2.17, 2.6, 2.85; .58, .68, .75, 1.1, 1.38, 1.77, 2.27, 2.7] V  diode_TjVec=[25, 125] degC  diode_VfVec=[.5, .7, .9, 1.3, 1.7, 2.1, 2.5] V  diode_IfVec=[.1, .2, .5, 1, 2, 4, 7, 10] A  diode_IrMat=[1e-06, 2e-06, 5e-06, 1e-05, 2.5e-05, 5e-05, .0001; 2e-06, 5e-06, 1e-05, 4e-05, 8e-05, .0002, .0005] A  diode_VrMat=[10, 100, 200, 250, 300, 325, 350; 10, 70, 160, 220, 270, 300, 320] V  diode_VrVec=[10, 20, 40, 50, 70, 80, 100] V  diode_IrVec=[1e-06, 2e-06, 5e-06, 1e-05, 2e-05, 5e-05, .0001] A  diode_Vr=-600 V  diode_Ls=150 nH  diode_Erec=0.03 J  diode_rec_loss_model=ee.enum.diode.reverseRecoveryModel.fixed  diode_ErecVal=0 J  diode_scaleWithIandV=true  diode_ErecMat=zeros(2, 3) J  diode_TjrecVec=[298.15, 398.15] K  diode_IfrecVec=[.1, 1, 10] A  diode_IrecVal=10 A  diode_VrecVal=10 V  diode_tFilter=1 / 1000 / 100 s  separateThermalPortForDiode=false  thermal_network_parameterization=ee.enum.thermalNetworkTopology.external  Rth=[.08, .5] K/W  Rth_Cauer=[.08, .1, .5] K/W  Rth_Foster=[.08, .14, .22, .16] K/W  thermal_mass_parameterization=ee.enum.thermalNetwork.timeconstant  thermal_mass=[.01, .5] J/K  thermal_mass_Cauer=[.01, .1, .5] J/K  thermal_mass_Foster=[.001, .005, .05, .5] J/K  thermal_time_constant=[.001, .2] s  thermal_time_constant_Cauer=[.001, .1, .2] s  thermal_time_constant_Foster=[7e-05, .0007, .01, .08] s  thermal_mass_initial_temperatures=[25, 25] degC  thermal_mass_initial_temperatures_Cauer=[25, 25, 25] degC  junction_thermal_mass=0.01 J/K  Tvec_initial_Foster=[25, 25, 25, 25] degC  RthDiode=[.03, .2] K/W  RthCauerDiode=[.03, .1, .2] K/W  RthFosterDiode=[.03, .2] K/W  thermalMassDiode=[3, 25] J/K  thermalMassCauerDiode=[3, 10, 25] J/K  thermalMassFosterDiode=[33, 50] J/K  thermalTauDiode=[.1, 5] s  thermalTauCauerDiode=[.1, 1, 5] s  thermalTauFosterDiode=[1, 10] s  thermalMassInitTempDiode=[25, 25] degC  thermalMassInitTempCauerDiode=[25, 25, 25] degC  junctionthermalMassDiode=0.1 J/K  TVecInitialFosterDiode=[25, 25, 25, 25] degC  no_thermal_network=0  IGBT_junction_temperature_specify=off  IGBT_junction_temperature_priority=None  IGBT_junction_temperature=25 degC  IGBT_junction_temperature_nominal_specify=off  IGBT_junction_temperature_nominal_value=1  IGBT_junction_temperature_nominal_unit=degC  diode_junction_temperature_specify=off  diode_junction_temperature_priority=None  diode_junction_temperature=25 degC  diode_junction_temperature_nominal_specify=off  diode_junction_temperature_nominal_value=1  diode_junction_temperature_nominal_unit=degC  Qj_specify=off  Qj_priority=None  Qj=0 W  Qj_nominal_specify=off  Qj_nominal_value=1  Qj_nominal_unit=W  accumulatedSwitchingLosses_specify=off  accumulatedSwitchingLosses_priority=None  accumulatedSwitchingLosses=0 J
  "IGBT (Ideal, Switching)2" : ee_lib/Semiconductors & Converters/IGBT (Ideal, Switching)  port_option=ee.enum.controlport.ps  Vf=0.8 V  Ron=0.001 Ohm  Goff=1e-5 1/Ohm  Vth=6 V  diode_param=ee.enum.semiconductors.protectionDiode.external  diode_Vf=0.8 V  diode_Ron=0.001 Ohm  diode_Goff=1e-5 1/Ohm  diode_C=50e-9 F  diode_iRM=-235 A  diode_iF=300 A  diode_idot=-50 A/us  diode_trr_param=ee.enum.converters.diodeReverseParam.trr_factor  diode_trr_factor=3  diode_trr=15 us  diode_Qrr=1500 s*uA  ice_specify=off  ice_priority=None  ice=0 A  ice_nominal_specify=off  ice_nominal_value=1  ice_nominal_unit=A  vce_specify=off  vce_priority=None  vce=0 V  vce_nominal_specify=off  vce_nominal_value=1  vce_nominal_unit=V  vge_specify=off  vge_priority=None  vge=0 V  vge_nominal_specify=off  vge_nominal_value=1  vge_nominal_unit=V  thermal_loss_option=ee.enum.converters.thermalLossOption.constantvalues  Von_data=[0, .1, .6, .8, 1, 1.3, 1.6, 2, 2.4; 0, .1, .7, 1, 1.2, 1.5, 1.9, 2.4, 2.8] V  Tj=[298.15, 398.15] K  Iout_data=[0, .1, 1, 5, 10, 20, 40, 70, 100] A  Eon_data=[0, .0024, .024, .12, .2, .48, 1.04, 2.16, 3.24; 0, .003, .03, .15, .25, .6, 1.3, 2.7, 4.05] * 1e-3 J  Eoff_data=[0, .0007, .0066, .033, .066, .17, .33, .83, 1.5; 0, .001, .01, .05, .1, .25, .5, 1.2, 2.2] * 1e-3 J  Eon_data_3D=[zeros(2, 9, 3)] J  Eoff_data_3D=[zeros(2, 9, 3)] J  Tj_loss=[298.15, 398.15] K  Iout_data_loss=[0, .1, 1, 5, 10, 20, 40, 70, 100] A  tabulateWithVce=false  Vce_loss=[0, 150, 300] V  Eon_scalar=22.86e-3 J  Eoff_scalar=17.14e-3 J  Voff=300 V  Iout_scalar=600 A  useCurrentFromPreviousCycle=false  useVoltageFromPreviousCycle=false  diodeModelType=ee.enum.converters.diodeModelType.pwl  diodeTableType=ee.enum.diode.tableType.IfMat  diode_ReverseIVType=ee.enum.diode.diodeReverseIV.constant  diode_IfMat=[.07, .12, .19, 1.75, 4.24, 7.32, 11.2; .16, .3, .72, 2.14, 4.02, 6.35, 9.12] A  diode_VfMat=[.9, 1.15, 1.25, 1.5, 1.75, 2.17, 2.6, 2.85; .58, .68, .75, 1.1, 1.38, 1.77, 2.27, 2.7] V  diode_TjVec=[25, 125] degC  diode_VfVec=[.5, .7, .9, 1.3, 1.7, 2.1, 2.5] V  diode_IfVec=[.1, .2, .5, 1, 2, 4, 7, 10] A  diode_IrMat=[1e-06, 2e-06, 5e-06, 1e-05, 2.5e-05, 5e-05, .0001; 2e-06, 5e-06, 1e-05, 4e-05, 8e-05, .0002, .0005] A  diode_VrMat=[10, 100, 200, 250, 300, 325, 350; 10, 70, 160, 220, 270, 300, 320] V  diode_VrVec=[10, 20, 40, 50, 70, 80, 100] V  diode_IrVec=[1e-06, 2e-06, 5e-06, 1e-05, 2e-05, 5e-05, .0001] A  diode_Vr=-600 V  diode_Ls=150 nH  diode_Erec=0.03 J  diode_rec_loss_model=ee.enum.diode.reverseRecoveryModel.fixed  diode_ErecVal=0 J  diode_scaleWithIandV=true  diode_ErecMat=zeros(2, 3) J  diode_TjrecVec=[298.15, 398.15] K  diode_IfrecVec=[.1, 1, 10] A  diode_IrecVal=10 A  diode_VrecVal=10 V  diode_tFilter=1 / 1000 / 100 s  separateThermalPortForDiode=false  thermal_network_parameterization=ee.enum.thermalNetworkTopology.external  Rth=[.08, .5] K/W  Rth_Cauer=[.08, .1, .5] K/W  Rth_Foster=[.08, .14, .22, .16] K/W  thermal_mass_parameterization=ee.enum.thermalNetwork.timeconstant  thermal_mass=[.01, .5] J/K  thermal_mass_Cauer=[.01, .1, .5] J/K  thermal_mass_Foster=[.001, .005, .05, .5] J/K  thermal_time_constant=[.001, .2] s  thermal_time_constant_Cauer=[.001, .1, .2] s  thermal_time_constant_Foster=[7e-05, .0007, .01, .08] s  thermal_mass_initial_temperatures=[25, 25] degC  thermal_mass_initial_temperatures_Cauer=[25, 25, 25] degC  junction_thermal_mass=0.01 J/K  Tvec_initial_Foster=[25, 25, 25, 25] degC  RthDiode=[.03, .2] K/W  RthCauerDiode=[.03, .1, .2] K/W  RthFosterDiode=[.03, .2] K/W  thermalMassDiode=[3, 25] J/K  thermalMassCauerDiode=[3, 10, 25] J/K  thermalMassFosterDiode=[33, 50] J/K  thermalTauDiode=[.1, 5] s  thermalTauCauerDiode=[.1, 1, 5] s  thermalTauFosterDiode=[1, 10] s  thermalMassInitTempDiode=[25, 25] degC  thermalMassInitTempCauerDiode=[25, 25, 25] degC  junctionthermalMassDiode=0.1 J/K  TVecInitialFosterDiode=[25, 25, 25, 25] degC  no_thermal_network=0  IGBT_junction_temperature_specify=off  IGBT_junction_temperature_priority=None  IGBT_junction_temperature=25 degC  IGBT_junction_temperature_nominal_specify=off  IGBT_junction_temperature_nominal_value=1  IGBT_junction_temperature_nominal_unit=degC  diode_junction_temperature_specify=off  diode_junction_temperature_priority=None  diode_junction_temperature=25 degC  diode_junction_temperature_nominal_specify=off  diode_junction_temperature_nominal_value=1  diode_junction_temperature_nominal_unit=degC  Qj_specify=off  Qj_priority=None  Qj=0 W  Qj_nominal_specify=off  Qj_nominal_value=1  Qj_nominal_unit=W  accumulatedSwitchingLosses_specify=off  accumulatedSwitchingLosses_priority=None  accumulatedSwitchingLosses=0 J
  Simulink-PS Converter1 : nesl_utility/Simulink-PS Converter  PhysicalDomain=network_engine_domain  SubClassName=ps_input  LeftPortType=input  RightPortType=output  PseudoPeriodic=off  Frequencies=[]  NoiseDistribution=none  NoiseParameters=[]  Unit=1  AffineConversion=off  FilteringAndDerivatives=provide  SimscapeFilterOrder=1  InputFilterTimeConstant=0.001  UdotUserProvided=0
  Simulink-PS Converter2 : nesl_utility/Simulink-PS Converter  PhysicalDomain=network_engine_domain  SubClassName=ps_input  LeftPortType=input  RightPortType=output  PseudoPeriodic=off  Frequencies=[]  NoiseDistribution=none  NoiseParameters=[]  Unit=1  AffineConversion=off  FilteringAndDerivatives=provide  SimscapeFilterOrder=1  InputFilterTimeConstant=0.001  UdotUserProvided=0
  Vcci : PMIOPort  Side=Left
  Vsi : PMIOPort  Port=2  Side=Left
  Vddi : PMIOPort  Port=3  Side=Left
  Vcco : PMIOPort  Port=4  Side=Right
  Vso : PMIOPort  Port=5  Side=Right
  Vddo : PMIOPort  Port=6  Side=Right
  wires:
  swh/1 -> Simulink-PS Converter2/1
  swl/1 -> Simulink-PS Converter1/1
  connections:
  Diode1/RConn1 -- Vcco/RConn1 -- Vcci/RConn1 -- "IGBT (Ideal, Switching)1"/RConn1
  Simulink-PS Converter2/RConn1 -- "IGBT (Ideal, Switching)1"/LConn1
  "IGBT (Ideal, Switching)1"/RConn2 -- Vso/RConn1 -- Vsi/RConn1 -- "IGBT (Ideal, Switching)2"/RConn1 -- Diode2/RConn1 -- Diode1/LConn1
  "IGBT (Ideal, Switching)2"/RConn2 -- Vddo/RConn1 -- Vddi/RConn1 -- Diode2/LConn1
  Simulink-PS Converter1/RConn1 -- "IGBT (Ideal, Switching)2"/LConn1
